simulink model "simulink_scheme_task_11"  (R2023b)
settings: Solver=ode4  StartTime=0.0  StopTime=simulationParameters.T_sim  FixedStep=simulationParameters.T_integration  RelTol=1e-3
values from neighbouring files (symbols this model uses):
  Kd = 30    [main_task_11.m]    (also in main_task_12.m)
  Ki = 0.1    [main_task_11.m]    (also in main_task_12.m)
  Kp = 15    [main_task_11.m]    (also in main_task_12.m)
  patientParameters = loadPatientParameter(patientID)    [main_task_12.m]
  simulationParameters = loadSimulationParameter    [main_task_11.m]    (also in main_task_12.m)
  T = simulationParameters.Ts    [main_task_11.m]    (also in main_task_12.m)
undefined symbols (not defined in the file or in its folder): PIDcontroller
settings Model: Creator=william  LastModifiedBy=william
settings DataIOCC: ReturnWorkspaceOutputs=off
settings ConfigComp: CovBoundaryAbsTol=1.0e-5

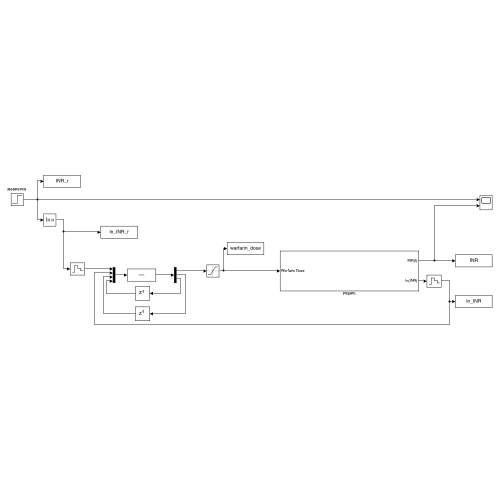
[thumbnail: Simulink's stored preview of the top-level diagram]
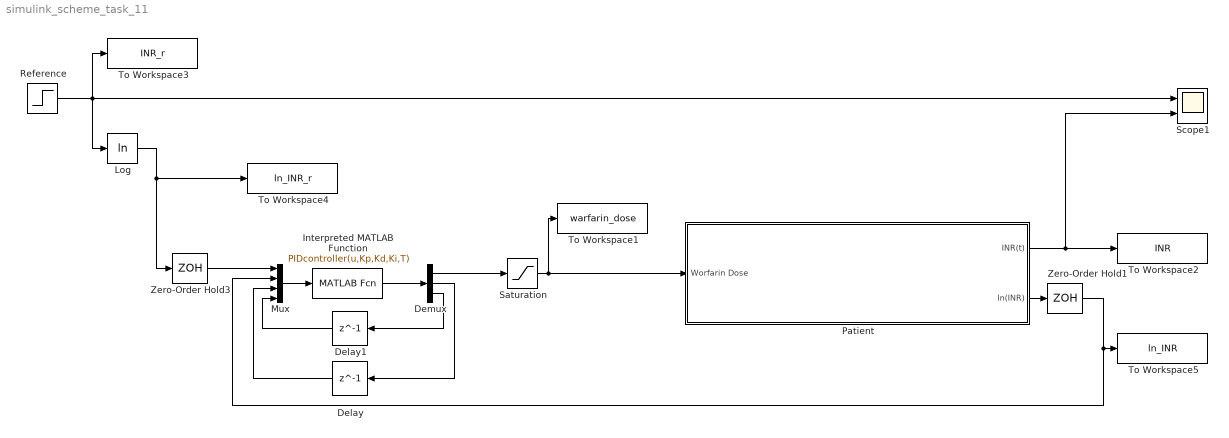
== system simulink_scheme_task_11 ==
  Delay : Delay  DelayLength=1  InitialCondition=0
  Delay1 : Delay  DelayLength=1  InitialCondition=0
  Demux : Demux  Outputs=3
  Interpreted MATLAB Function : MATLABFcn  MATLABFcn=PIDcontroller(u,Kp,Kd,Ki,T)  OutputDimensions=3
  Log : Math  Operator=log
  Mux : Mux
  Patient : Subsystem
  Reference : Step  Time=2*24  Before=1  After=2.5  SampleTime=simulationParameters.Ts
  Saturation : Saturate  UpperLimit=simulationParameters.u_max  LowerLimit=simulationParameters.u_min
  Scope1 : Scope  NumInputPorts=2
  To Workspace1 : ToWorkspace  VariableName=warfarin_dose  SaveFormat=Structure With Time  SampleTime=-1
  To Workspace2 : ToWorkspace  VariableName=INR  SaveFormat=Structure With Time  SampleTime=-1
  To Workspace3 : ToWorkspace  VariableName=INR_r  SaveFormat=Structure With Time  SampleTime=-1
  To Workspace4 : ToWorkspace  VariableName=ln_INR_r  SaveFormat=Structure With Time  SampleTime=-1
  To Workspace5 : ToWorkspace  VariableName=ln_INR  SaveFormat=Structure With Time  SampleTime=-1
  Zero-Order Hold1 : ZeroOrderHold  SampleTime=simulationParameters.Ts
  Zero-Order Hold3 : ZeroOrderHold  SampleTime=simulationParameters.Ts
  wires:
  Saturation/1 -> To Workspace1/1, Patient/1(Worfarin Dose)
  Demux/2 -> Delay/1
  Delay/1 -> Mux/3
  Demux/1 -> Saturation/1
  Patient/1(INR(t)) -> Scope1/2, To Workspace2/1
  Zero-Order Hold3/1 -> Mux/1
  Demux/3 -> Delay1/1
  Log/1 -> To Workspace4/1, Zero-Order Hold3/1
  Mux/1 -> Interpreted MATLAB Function/1
  Patient/2(ln(INR)) -> Zero-Order Hold1/1
  Reference/1 -> To Workspace3/1, Log/1, Scope1/1
  Delay1/1 -> Mux/4
  Zero-Order Hold1/1 -> Mux/2, To Workspace5/1
  Interpreted MATLAB Function/1 -> Demux/1

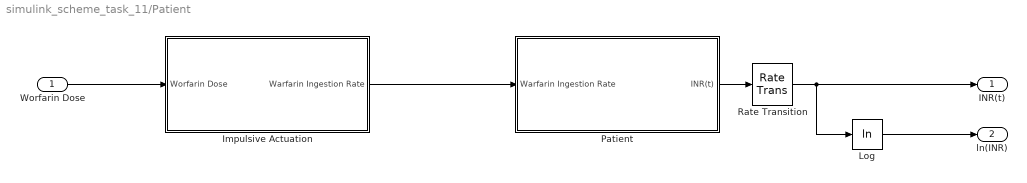
== system simulink_scheme_task_11/Patient ==
  Worfarin Dose : Inport
  Impulsive Actuation : Subsystem
  Log : Math  Operator=log
  Patient : Subsystem
  Rate Transition : RateTransition  InitialCondition=patientParameters.BASE  OutPortSampleTime=simulationParameters.Ts
  INR(t) : Outport
  ln(INR) : Outport  Port=2
  wires:
  Rate Transition/1 -> INR(t)/1, Log/1
  Worfarin Dose/1 -> Impulsive Actuation/1(Worfarin Dose)
  Impulsive Actuation/1(Warfarin Ingestion Rate) -> Patient/1("Warfarin Ingestion Rate ")
  Patient/1(INR(t)) -> Rate Transition/1
  Log/1 -> ln(INR)/1

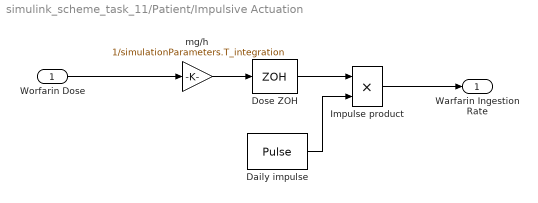
== system simulink_scheme_task_11/Patient/Impulsive Actuation ==
  Worfarin Dose : Inport
  Daily impulse : DiscretePulseGenerator  Period=simulationParameters.Ts/simulationParameters.T_integration  SampleTime=simulationParameters.T_integration
  Dose ZOH : ZeroOrderHold  SampleTime=simulationParameters.T_integration
  Impulse product : Product  Inputs=**
  mg/h : Gain  Gain=1/simulationParameters.T_integration
  Warfarin Ingestion Rate : Outport
  wires:
  Worfarin Dose/1 -> mg/h/1
  mg/h/1 -> Dose ZOH/1
  Dose ZOH/1 -> Impulse product/1
  Daily impulse/1 -> Impulse product/2
  Impulse product/1 -> Warfarin Ingestion Rate/1

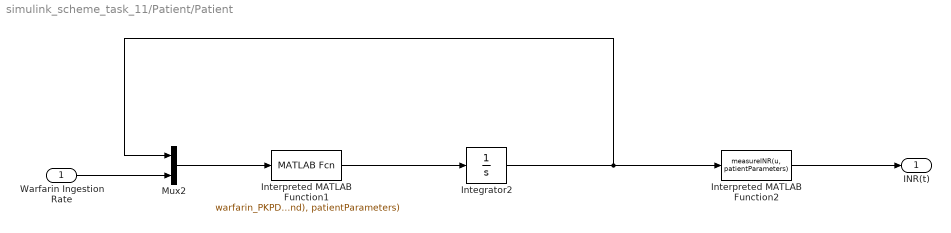
== system simulink_scheme_task_11/Patient/Patient ==
  "Warfarin Ingestion Rate " : Inport
  Integrator2 : Integrator  InitialCondition=[patientParameters.x0,patientParameters.appearance.x0]
  Interpreted MATLAB Function1 : MATLABFcn  MATLABFcn=warfarin_PKPD_model(u(1:end-1), u(end), patientParameters)  OutputDimensions=8
  Interpreted MATLAB Function2 : MATLABFcn  MATLABFcn=measureINR(u, patientParameters)
  Mux2 : Mux  Inputs=2
  INR(t) : Outport
  wires:
  Interpreted MATLAB Function1/1 -> Integrator2/1
  Interpreted MATLAB Function2/1 -> INR(t)/1
  Integrator2/1 -> Mux2/1, Interpreted MATLAB Function2/1
  Mux2/1 -> Interpreted MATLAB Function1/1
  "Warfarin Ingestion Rate "/1 -> Mux2/2
